simulink model "usv_heading_pid"  (R2024b)
settings: Solver=ode4  StartTime=0  StopTime=300  FixedStep=0.01  RelTol=1e-3
settings Model: Creator=qianr  LastModifiedBy=qianr
settings DataIOCC: SaveOutput=off  SignalLogging=off  SaveTime=off  ReturnWorkspaceOutputs=off

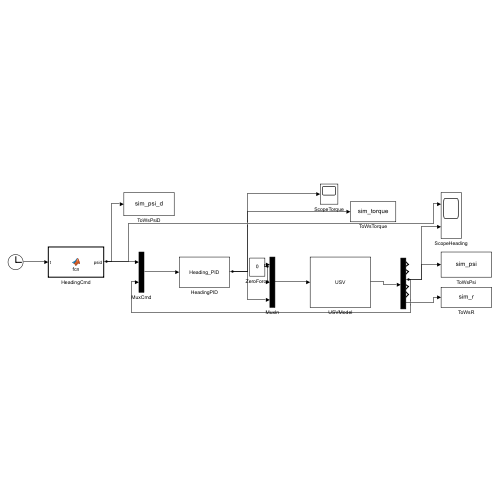
[thumbnail: Simulink's stored preview of the top-level diagram]
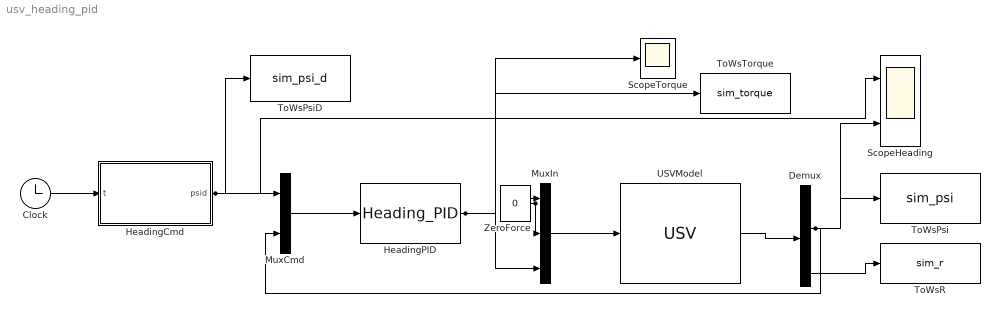
== system usv_heading_pid ==
  Clock : Clock
  Demux : Demux  Outputs=6
  HeadingCmd : MATLAB Function  TreatAsAtomicUnit=on
  HeadingPID : S-Function  FunctionName=Heading_PID  Parameters=cfg_pid  SFunctionDeploymentMode=off  EnableBusSupport=off
  MuxCmd : Mux  Inputs=2
  MuxIn : Mux  Inputs=3
  ScopeHeading : Scope  NumInputPorts=2
  ScopeTorque : Scope
  ToWsPsi : ToWorkspace  VariableName=sim_psi  SaveFormat=Timeseries  SampleTime=0.01
  ToWsPsiD : ToWorkspace  VariableName=sim_psi_d  SaveFormat=Timeseries  SampleTime=0.01
  ToWsR : ToWorkspace  VariableName=sim_r  SaveFormat=Timeseries  SampleTime=0.01
  ToWsTorque : ToWorkspace  VariableName=sim_torque  SaveFormat=Timeseries  SampleTime=0.01
  USVModel : S-Function  FunctionName=USV  Parameters=cfg_usv  SFunctionDeploymentMode=off  EnableBusSupport=off
  ZeroForce : Constant  Value=0
  wires:
  Clock/1 -> HeadingCmd/1(t)
  HeadingCmd/1(psid) -> MuxCmd/1, ScopeHeading/1, ToWsPsiD/1
  Demux/3 -> MuxCmd/2, ScopeHeading/2, ToWsPsi/1
  MuxCmd/1 -> HeadingPID/1
  HeadingPID/1 -> MuxIn/3, ScopeTorque/1, ToWsTorque/1
  ZeroForce/1 -> MuxIn/1, MuxIn/2
  MuxIn/1 -> USVModel/1
  USVModel/1 -> Demux/1
  Demux/6 -> ToWsR/1

== matlab function usv_heading_pid/HeadingCmd ==
  data: t input; psid output
function psid = fcn(t)
%#codegen
if t < 42
    psid = 30*pi/180;
elseif t < 104
    psid = 230*pi/180;
else
    psid = 30*pi/180;
end
